simulink model "impmodel"  (R2023a)
settings: Solver=FixedStepDiscrete  StartTime=0.0  StopTime=8  RelTol=1e-3  EnableMultiTasking=on
values from neighbouring files (symbols this model uses):
  availableSpeedModes = 3    [params_f2838.mat]
  inverter_DRV8300 =     [params_f2838.mat]
  PI_params =     [params_f2838.mat]
  pmsm_ECI6360 =     [params_f2838.mat]
  PU_System =     [params_f2838.mat]
  target_f2838 =     [params_f2838.mat]
  Ts = 5e-05    [params_f2838.mat]
  Ts_motor = 2.5e-05    [params_f2838.mat]
  Ts_simulink = 2.5e-05    [params_f2838.mat]
  Ts_speed = 0.0005    [params_f2838.mat]
undefined symbols (not defined in the file or in its folder): Down, GPTRIP1SEL, TZ1, Up
libraries: simulink x35, c2802xlib x11, idelinklib_common x8, procinterlib x8, mcbcontrolslib x8, c280xlib x7, mcbpositiondecoderlib x7, slpidlib x5, svdschedulerlib x4, c2838xlib x2, autolibpmsminterior x1, mcbplantlib x1
(part 4 of 4)

== system impmodel/Torque Controller/Input Scaling/CodeGeneration/Calculate Position from Hall/Atomic Hall Reading/Subsystem1 ==
  function-call : TriggerPort  TriggerType=function-call  VariantControl=(inherit)  PortDimensions=1
  Memory Copy : idelinklib_common/Memory Copy  copyFrom=Specified source code symbol  copyFromAddressSource=Specify via dialog  copyFromAddress=hex2dec('00001000')  copyFromSrcCode=&ECap1Regs.TSCTR  dataTypeFrom=uint32  dataDimensionFrom=1  useOffsetFrom=off  offsetFromSrc=Specify via dialog  offsetFrom=0  strideFrom=1  copyTo=Output port  copyToAddressSource=Specify via dialog  copyToAddress=hex2dec('00002000')  copyToSrcCode=myVariableDst  dataTypeTo=uint32  useOffsetTo=off  offsetToSrc=Specify via dialog  offsetTo=0  strideTo=1  sampleTime=-1  useInitValue=off  initValueSrc=Specify constant value  initValue=1  initValueSrcCode=myInitValueVariable  useAsMask=off  maskOperator=bitwise AND  useTermValue=off  termValue=1  isRealtimeEnabled=off  emitCCBeforeWrite=off  CCBeforeWrite=/* Custom Code Before Write*/  emitCCAfterWrite=off  CCAfterWrite=/* Custom Code After Write*/
  Memory Copy1 : idelinklib_common/Memory Copy  copyFrom=Specified source code symbol  copyFromAddressSource=Specify via dialog  copyFromAddress=hex2dec('00001000')  copyFromSrcCode=&ECap2Regs.TSCTR  dataTypeFrom=uint32  dataDimensionFrom=1  useOffsetFrom=off  offsetFromSrc=Specify via dialog  offsetFrom=0  strideFrom=1  copyTo=Output port  copyToAddressSource=Specify via dialog  copyToAddress=hex2dec('00002000')  copyToSrcCode=myVariableDst  dataTypeTo=uint32  useOffsetTo=off  offsetToSrc=Specify via dialog  offsetTo=0  strideTo=1  sampleTime=-1  useInitValue=off  initValueSrc=Specify constant value  initValue=1  initValueSrcCode=myInitValueVariable  useAsMask=off  maskOperator=bitwise AND  useTermValue=off  termValue=1  isRealtimeEnabled=off  emitCCBeforeWrite=off  CCBeforeWrite=/* Custom Code Before Write*/  emitCCAfterWrite=off  CCAfterWrite=/* Custom Code After Write*/
  Memory Copy2 : idelinklib_common/Memory Copy  copyFrom=Specified source code symbol  copyFromAddressSource=Specify via dialog  copyFromAddress=hex2dec('00001000')  copyFromSrcCode=&ECap3Regs.TSCTR  dataTypeFrom=uint32  dataDimensionFrom=1  useOffsetFrom=off  offsetFromSrc=Specify via dialog  offsetFrom=0  strideFrom=1  copyTo=Output port  copyToAddressSource=Specify via dialog  copyToAddress=hex2dec('00002000')  copyToSrcCode=myVariableDst  dataTypeTo=uint32  useOffsetTo=off  offsetToSrc=Specify via dialog  offsetTo=0  strideTo=1  sampleTime=-1  useInitValue=off  initValueSrc=Specify constant value  initValue=1  initValueSrcCode=myInitValueVariable  useAsMask=off  maskOperator=bitwise AND  useTermValue=off  termValue=1  isRealtimeEnabled=off  emitCCBeforeWrite=off  CCBeforeWrite=/* Custom Code Before Write*/  emitCCAfterWrite=off  CCAfterWrite=/* Custom Code After Write*/
  Min : MinMax  Inputs=3
  CounterIn : Outport
  wires:
  Memory Copy1/1 -> Min/2
  Min/1 -> CounterIn/1
  Memory Copy/1 -> Min/1
  Memory Copy2/1 -> Min/3

== system impmodel/Torque Controller/Input Scaling/CodeGeneration/Calculate Position from Hall/Atomic Hall Reading/Integrity_Check/No_Integrity_issue ==
  Counter : Inport
  Action Port : ActionPort  ActionPortLabel=if(u1 == 0)
  Out1 : Outport
  wires:
  Counter/1 -> Out1/1

== system impmodel/Torque Controller/Input Scaling/CodeGeneration/Calculate Position from Hall/Atomic Hall Reading/Integrity_Check/Refresh_Halls ==
  Action Port : ActionPort  ActionPortLabel=else
  Bitwise OR : simulink/Logic and Bit Operations/Bitwise Operator  logicop=OR  UseBitMask=off  NumInputPorts=3  BitMask=bin2dec('11011001')  BitMaskRealWorld=Stored Integer
      settings: LibrarySourceBlock=|
      | simulink/Quick Insert/Logic and Bit
      | Operations/Bitwise OR
  Data Type Conversion : DataTypeConversion  OutDataTypeStr=uint32  ConvertRealWorld=Stored Integer (SI)  SaturateOnIntegerOverflow=off  RndMeth=Floor
  GPIO 24 Hall_A : simulink/Logic and Bit Operations/Bitwise Operator  logicop=AND  UseBitMask=on  BitMask=hex2dec('1000000')  BitMaskRealWorld=Stored Integer
      settings: LibrarySourceBlock=|
      | simulink/Quick Insert/Logic and Bit
      | Operations/Bitwise AND
  GPIO 25 Hall_B : simulink/Logic and Bit Operations/Bitwise Operator  logicop=AND  UseBitMask=on  BitMask=hex2dec('2000000')  BitMaskRealWorld=Stored Integer
      settings: LibrarySourceBlock=|
      | simulink/Quick Insert/Logic and Bit
      | Operations/Bitwise AND
  GPIO 26 Hall_C : simulink/Logic and Bit Operations/Bitwise Operator  logicop=AND  UseBitMask=on  BitMask=hex2dec('4000000')  BitMaskRealWorld=Stored Integer
      settings: LibrarySourceBlock=|
      | simulink/Quick Insert/Logic and Bit
      | Operations/Bitwise AND
  Memory Copy : idelinklib_common/Memory Copy  copyFrom=Specified source code symbol  copyFromAddressSource=Specify via dialog  copyFromAddress=hex2dec('00001000')  copyFromSrcCode=&GpioDataRegs.GPADAT.all  dataTypeFrom=uint32  dataDimensionFrom=1  useOffsetFrom=off  offsetFromSrc=Specify via dialog  offsetFrom=0  strideFrom=1  copyTo=Output port  copyToAddressSource=Specify via dialog  copyToAddress=hex2dec('00002000')  copyToSrcCode=myVariableDst  dataTypeTo=uint32  useOffsetTo=off  offsetToSrc=Specify via dialog  offsetTo=0  strideTo=1  sampleTime=-1  useInitValue=off  initValueSrc=Specify constant value  initValue=1  initValueSrcCode=myInitValueVariable  useAsMask=off  maskOperator=bitwise AND  useTermValue=off  termValue=1  isRealtimeEnabled=off  emitCCBeforeWrite=off  CCBeforeWrite=/* Custom Code Before Write*/  emitCCAfterWrite=off  CCAfterWrite=/* Custom Code After Write*/
  Shift Arithmetic : ArithShift  BitShiftNumber=26
  Shift Arithmetic1 : ArithShift  BitShiftNumber=24
  Shift Arithmetic2 : ArithShift  BitShiftNumber=22
  Out1 : Outport
  wires:
  Data Type Conversion/1 -> Out1/1
  Shift Arithmetic2/1 -> Bitwise OR/3
  Shift Arithmetic1/1 -> Bitwise OR/2
  GPIO 25 Hall_B/1 -> Shift Arithmetic1/1
  Memory Copy/1 -> GPIO 26 Hall_C/1, GPIO 24 Hall_A/1, GPIO 25 Hall_B/1
  Shift Arithmetic/1 -> Bitwise OR/1
  Bitwise OR/1 -> Data Type Conversion/1
  GPIO 24 Hall_A/1 -> Shift Arithmetic2/1
  GPIO 26 Hall_C/1 -> Shift Arithmetic/1
